simulink model "lab_04_mdl_22a"  (R2022a)
settings: Solver=FixedStepAuto  StartTime=0.0  StopTime=200  FixedStep=10  RelTol=1e-3
undefined symbols (not defined in the file or in its folder): DiscIntNeverNeededParam
settings Model: Creator=User  LastModifiedBy=salgi
settings ModelReferenceCC: EnableRefExpFcnMdlSchedulingChecks=off
settings RTWCC: Description=Generic Real-Time Target

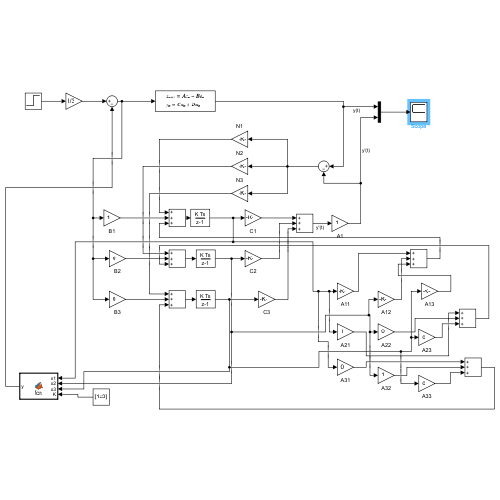
[thumbnail: Simulink's stored preview of the top-level diagram]
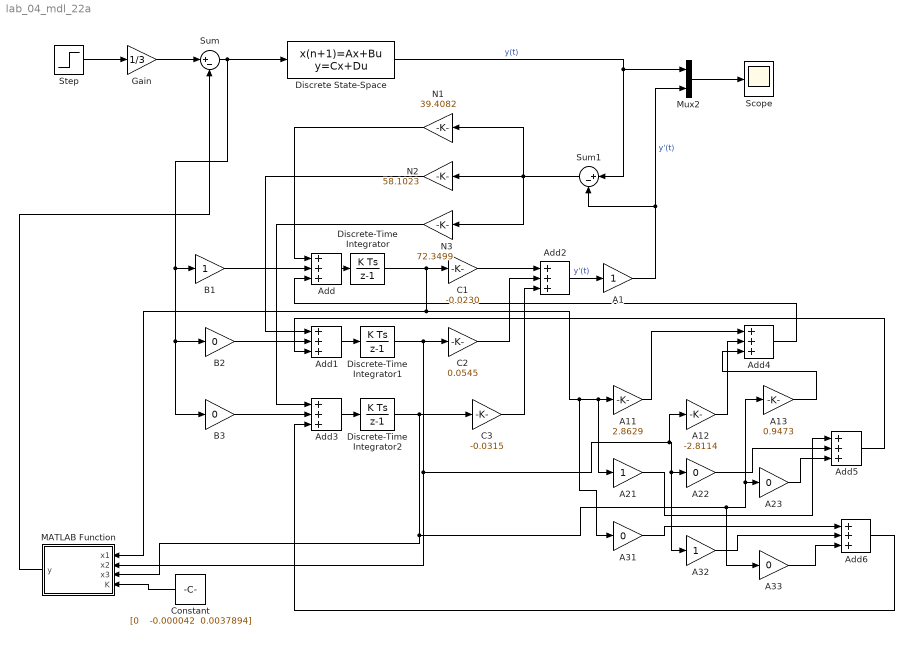
== system lab_04_mdl_22a ==
  A33 : Gain  Gain=0
  Add{,1..6} (7 alike) : Sum  Inputs=+++
  B1 : Gain
  B2 : Gain  Gain=0
  B3 : Gain  Gain=0
  C1 : Gain  Gain=-0.0230
  C2 : Gain  Gain=0.0545
  C3 : Gain  Gain=-0.0315
  Constant : Constant  Value="[0    -0.000042  0.0037894]"
  Discrete State-Space : DiscreteStateSpace  A="[2.8629   -2.8114    0.9473;0 1 0; 0 0 1]"  B=[1; 0; 0]  C="[-0.0230    0.0545   -0.0315]"  D=1.006  SampleTime=-1
  Discrete-Time Integrator : DiscreteIntegrator  InitialCondition=1  SampleTime=-1  ICPrevOutput=DiscIntNeverNeededParam  ICPrevScaledInput=DiscIntNeverNeededParam
  Discrete-Time Integrator1 : DiscreteIntegrator  InitialCondition=2  SampleTime=-1  ICPrevOutput=DiscIntNeverNeededParam  ICPrevScaledInput=DiscIntNeverNeededParam
  Discrete-Time Integrator2 : DiscreteIntegrator  InitialCondition=1  SampleTime=-1  ICPrevOutput=DiscIntNeverNeededParam  ICPrevScaledInput=DiscIntNeverNeededParam
  Gain : Gain  Gain=1/3
  MATLAB Function : MATLAB Function  TreatAsAtomicUnit=on
  Mux2 : Mux  Inputs=2
  N1 : Gain  Gain=39.4082
  N2 : Gain  Gain=58.1023
  N3 : Gain  Gain=72.3499
  Scope : Scope
  Step : Step  SampleTime=0.1
  Sum : Sum  Inputs=|+-
  Sum1 : Sum  Inputs=|+-
  А1 : Gain
  А11 : Gain  Gain=2.8629
  А12 : Gain  Gain=-2.8114
  А13 : Gain  Gain=0.9473
  А21 : Gain
  А22 : Gain  Gain=0
  А23 : Gain  Gain=0
  А31 : Gain  Gain=0
  А32 : Gain
  wires:
  Step/1 -> Gain/1
  Gain/1 -> Sum/1
  Sum/1 -> B3/1, B2/1, B1/1, Discrete State-Space/1
  Discrete State-Space/1 -> Mux2/1, Sum1/1  "y(t)"
  N2/1 -> Add1/1
  B1/1 -> Add/2
  B2/1 -> Add1/2
  Add/1 -> Discrete-Time Integrator/1
  Add1/1 -> Discrete-Time Integrator1/1
  Discrete-Time Integrator/1 -> MATLAB Function/1(x1), А31/1, А21/1, А11/1, C1/1
  C1/1 -> Add2/1
  Discrete-Time Integrator1/1 -> MATLAB Function/2(x2), А32/1, А22/1, А12/1, C2/1
  N1/1 -> Add/1
  N3/1 -> Add3/1
  B3/1 -> Add3/2
  Add3/1 -> Discrete-Time Integrator2/1
  Discrete-Time Integrator2/1 -> MATLAB Function/3(x3), А23/1, А13/1, A33/1, C3/1
  C2/1 -> Add2/2
  C3/1 -> Add2/3
  Add4/1 -> Add/3
  А11/1 -> Add4/1
  А12/1 -> Add4/2
  А13/1 -> Add4/3
  А21/1 -> Add5/1
  А22/1 -> Add5/2
  А23/1 -> Add5/3
  Add5/1 -> Add1/3
  A33/1 -> Add6/3
  А32/1 -> Add6/2
  А31/1 -> Add6/1
  Add6/1 -> Add3/3
  MATLAB Function/1(y) -> Sum/2
  Sum1/1 -> N1/1, N3/1, N2/1
  Mux2/1 -> Scope/1
  Constant/1 -> MATLAB Function/4(K)
  Add2/1 -> А1/1  "y'(t)"
  А1/1 -> Sum1/2, Mux2/2  "y'(t)"

== matlab function lab_04_mdl_22a/MATLAB Function ==
  data: x1 input; y output; x2 input; x3 input; K input
function y = fcn(x1,x2,x3,K)

y = K(1)*x1 + K(2)*x2+K(3)*x3;
